simulink model "hdlcoder_ofdm_fft_eml"  (R2026a)
settings: Solver=FixedStepDiscrete  StopTime=5000
PreLoadFcn:
  | wordLength = 12;
  | fracLength = 6;
InitFcn:
  | TotalPoint= 512;
  | TotalStage= 9;
  | FFT_nt=numerictype(1,12, 6);
  | twiddle_Signed = 1;
  | twiddle_WordLength = 12;
  | twiddle_FractionLength = 10;
  | twiddle_nt=numerictype(1,12, 10);
undefined symbols (not defined in the file or in its folder): EbNodB, M, Tsym
libraries: hdlsllib x10, commdigbbndam3 x3, dspxfrm3 x2, commsink2 x2, commchan3 x1, simulink x1, commseqgen3 x1, dspindex x1, commrandsrc3 x1
(part 3 of 3)

== matlab function hdlcoder_ofdm_fft_eml/FFT_512Pt_EML_Serial/Serialized_FFT/FFT_Stages/FFT_Stage9/Control_Logic ==
  settings: fimath=hdlfimath
  data: fft2_x input FFT_nt; fft2_y input FFT_nt; fft2_u output FFT_nt; fft2_v output FFT_nt; twiddle_addr output; enable input boolean; data_in input FFT_nt; index_in input fixdt(0,TotalStage+1,0); data_en output boolean; data_out output FFT_nt; index_out output; mem_rd_dout input FFT_nt; mem_wr_din output FFT_nt; mem_wr_addr output; mem_wr_en output; mem_rd_addr output; TotalStage parameter
function [fft2_u, fft2_v, twiddle_addr, data_en, data_out, index_out, mem_wr_din, mem_wr_addr, mem_wr_en, mem_rd_addr] ...
          = fcn(fft2_x, fft2_y, enable, data_in, index_in, mem_rd_dout, TotalStage)
% FF2 Stages in Serial FFT Model
% Each stage is composed of one FFT2 butterfly computing unit, 
% some memory to cache the streaming data and twiddles, and some control logics.
%
% The incoming streaming data are first stored into cache memory in the data order of last stage,
% and then they are read out in the data order of current stage and send to FFT computing unit.
% The computing unit will produce one result data every clock cycle, and the data_out will streaming
% out the result data in the order of current stage.
% 
% The memory size of each stage is the same as Stage Number, except Stage 1 (the minimum size of
% the memory block is 2). So all the stages share the same code except Stage 1.
% 
% To expand the size of FFT model, user can simply copy and paste new stage blocks and insert them
% before the End_Stage_Reorder block. Only the "Stage" in this code needs to be modified in the new block. 
% And also the size of memory blocks needs to be modified in the new block.
      
Stage = 9;      

N = uint16(2^(Stage-1));
nt = numerictype(data_in);
fm = fimath(data_in);

nt1 = numerictype(0, Stage+1, 0);
nt2 = numerictype(0, Stage-1, 0);
nt3 = numerictype(0, TotalStage-Stage+1, 0);
nt_addr = numerictype(0, TotalStage+1, 0);

% State machine registers
persistent main_state butterfly_state 
nts = numerictype(0, 2, 0);
if isempty(main_state)
    main_state = getfi(0, nts);
end
if isempty(butterfly_state)
    butterfly_state = getfi(0, nts);
end

% Address counters
persistent mem_addr mem_addr1 mem_addr2 
if isempty(mem_addr)
    mem_addr  = getfi(0, nt_addr);
end
if isempty(mem_addr1)
    mem_addr1 = getfi(0, nt_addr);
end
if isempty(mem_addr2)
    mem_addr2 = getfi(0, nt_addr);
end

persistent ctr ctr_lsb1c ctr_lsb2c ctr_msb
if isempty(ctr)
    ctr       = getfi(0, nt1);
end
if isempty(ctr_lsb1c)
    ctr_lsb1c = getfi(0, nt2);
end
if isempty(ctr_lsb2c)
    ctr_lsb2c = getfi(0, nt2);
end
if isempty(ctr_msb)
    ctr_msb   = getfi(0, nt3);
end

% Input/Output
mem_rd_addr  = bitsliceget(mem_addr, Stage, 1);
mem_wr_addr  = bitsliceget(index_in, Stage, 1);
mem_wr_din   = data_in;
index_out    = mem_addr;
twiddle_addr = ctr_lsb1c;

% Delay register inserted before the FFT2 computing unit
persistent reg_u reg_v
if isempty(reg_u)
    reg_u = complex(getfi(0, nt));
end
if isempty(reg_v)
    reg_v = complex(getfi(0, nt));
end
fft2_u = reg_u;
fft2_v = reg_v;

% Main state machine control the memory and data enable signals
switch uint8(main_state)
    case 0 %initial
        mem_wr_en    = false;
        calcu_en     = false;
        data_en      = false;
        ctr_en       = false;
        if enable
            main_state = getfi(1, nts);
        else
            main_state = getfi(0, nts);
        end
        
    case 1 %write data
        mem_wr_en    = true;
        calcu_en     = false;
        data_en      = false;
        ctr_en       = true;
        if ctr == getfi(N-2, nt1)
            main_state = getfi(2, nts);
        else
            main_state = getfi(1, nts);
        end
       
    case 2 %read & calculate data
        mem_wr_en    = true;
        calcu_en     = true;
        data_en      = false;
        ctr_en       = true;
        if ctr == getfi(N+4, nt1)
            main_state = getfi(3, nts);
        else
            main_state = getfi(2, nts);
        end

    case 3 %set output data_en signal, keep calculation
        mem_wr_en    = true;
        calcu_en     = true;
        data_en      = true;
        ctr_en       = false;
        main_state   = getfi(3, nts);
        
    otherwise
        mem_wr_en    = false;
        calcu_en     = false;
        data_en      = false;
        ctr_en       = false;
        main_state   = getfi(0, nts);
end

% Butterfly calculation state machine controls the memory access and data movement
switch uint8(butterfly_state)
    case 0 %initial
        data_out    = fft2_x;
        mem_addr    = mem_addr1;
        ctr_lsb1_en = false;
        ctr_lsb2_en = false;        
        if calcu_en
            butterfly_state = getfi(1, nts);
        else
            butterfly_state = getfi(0, nts);
        end
        
    case 1 %pre-read data
        data_out    = fft2_y;    
        mem_addr    = mem_addr2;
        ctr_lsb1_en = true;
        ctr_lsb2_en = false;
        butterfly_state = getfi(2, nts);

    case 2 %read data -> reg_u
        reg_u       = mem_rd_dout;
        data_out    = fft2_y;
        mem_addr    = mem_addr1;
        ctr_lsb1_en = false;
        ctr_lsb2_en = true;
        butterfly_state = getfi(3, nts);

    case 3 %read data -> reg_v
        reg_v       = mem_rd_dout;       
        data_out    = fft2_x;
        mem_addr    = mem_addr2;
        ctr_lsb1_en = true;
        ctr_lsb2_en = false;
        butterfly_state = getfi(2, nts);   
        
    otherwise
        data_out    = fft2_y;
        mem_addr    = mem_addr1;
        ctr_lsb1_en = false;
        ctr_lsb2_en = false;
        butterfly_state = getfi(0, nts);
end

% Memory address msb counter enable signal
if (ctr_lsb1_en == true) && (ctr_lsb1c == getfi(N-1, nt2))
    ctr_msb_en = true;
else
    ctr_msb_en = false;
end

% Mem_count counter
ctr = update_counter(ctr_en, ctr, nt1);

% Memory address lsb counter 1 
ctr_lsb1c = update_counter(ctr_lsb1_en, ctr_lsb1c, nt2);

% Memory address lsb counter 2
ctr_lsb2c = update_counter(ctr_lsb2_en, ctr_lsb2c, nt2);

% Memory address msb counter
%ctr_msb = update_counter(ctr_msb_en, ctr_msb, nt3);
if ctr_msb_en
    if ctr_msb == getfi(0, nt3)
        ctr_msb = getfi(1, nt3);
    else
        ctr_msb = getfi(0, nt3);
    end    
end

% The output address representation
c0_ufix1 = fi(0, 0, 1, 0, fm);
c1_ufix1 = fi(1, 0, 1, 0, fm);
ctr_lsb1 = bitconcat(c0_ufix1, ctr_lsb1c);
ctr_lsb2 = bitconcat(c1_ufix1, ctr_lsb2c);
mem_addr1 = bitconcat(ctr_msb, ctr_lsb1);
mem_addr2 = bitconcat(ctr_msb, ctr_lsb2);
                  
end

function out = update_counter(enable, in, nt)
if enable
    out = getfi(in + getfi(1, nt), nt);
else
    out = in;
end
end

function f = getfi(u, nt)
f = fi(u, nt, hdlfimath);
end

== matlab function hdlcoder_ofdm_fft_eml/FFT_512Pt_EML_Serial/Serialized_FFT/FFT_Stages/FFT_Stage9/Twiddle_ROM ==
  settings: fimath=hdlfimath
  data: twiddle_addr input; fft2_twiddle output twiddle_nt; TotalPoint parameter; twiddle_Signed parameter; twiddle_WordLength parameter; twiddle_FractionLength parameter
function fft2_twiddle = fcn(twiddle_addr, TotalPoint, twiddle_Signed, twiddle_WordLength, twiddle_FractionLength)
% Twiddle ROM

Stage = 9;

nt = numerictype(twiddle_Signed, twiddle_WordLength, twiddle_FractionLength);
fm = fimath(...
'RoundMode', 'nearest',...
'OverflowMode', 'saturate',...
'ProductMode', 'FullPrecision', 'ProductWordLength', 128,...
'SumMode', 'FullPrecision', 'SumWordLength', 128,...
'CastBeforeSum', true);

% Provide twiddle data for FFT calculation
persistent twiddleValue
if isempty(twiddleValue)
    twiddleValue = fi(exp(-2*pi*1i*(0:(TotalPoint/(2^Stage)):(TotalPoint/2-1))/TotalPoint).', nt, fm);   
end
fft2_twiddle = twiddleValue(int32(twiddle_addr)+1);

== matlab function hdlcoder_ofdm_fft_eml/FFT_512Pt_EML_Serial/Serialized_FFT/Start_Stage_BitReverse/BitReverse_Control_Logics ==
  settings: fimath=hdlfimath
  data: enable input boolean; data_in input FFT_nt; data_en output; data_out output; mem_rd_dout input FFT_nt; mem_wr_din output FFT_nt; mem_wr_addr output; mem_wr_en output; mem_rd_addr output; TotalPoint parameter; TotalStage parameter
function [data_en, data_out, mem_wr_din, mem_wr_addr, mem_wr_en, mem_rd_addr] ...
          = fcn(enable, data_in, mem_rd_dout, TotalPoint, TotalStage)
% Starting Stage -- Bitreverse the order of input serial data
% Memory sized as much as TotalPoint*2 are used to temporary cache the incoming data stream
% The initial delay of this block is fixed as TotalPoint
      
nt = numerictype(data_in);
nt_addr = numerictype(0, TotalStage+1, 0);

% State machines 
persistent main_state
nts = numerictype(0, 2, 0);
if isempty(main_state)
    main_state = getfi(0, nts);
end

% Memory address counters
persistent index_in mem_addr
if isempty(index_in)
    index_in = getfi(0, nt_addr);
end
if isempty(mem_addr)
    mem_addr = getfi(0, nt_addr);
end

% Input/Output
mem_rd_addr = mem_addr;
mem_wr_addr = bitconcat([bitget(index_in, TotalStage+1), bitget(index_in, 1:TotalStage)]);
data_out = mem_rd_dout;

% Delay register for data_in 
persistent reg_data_in
if isempty(reg_data_in)
    reg_data_in = complex(getfi(0, nt));
end

mem_wr_din  = reg_data_in;
reg_data_in = data_in;

switch uint8(main_state)
    case 0 %initial
        mem_wr_en   = false;
        index_in_en = false;
        data_en     = false;
        mem_addr_en = false;        
        if enable
            main_state = getfi(1, nts);
        else
            main_state = getfi(0, nts);
        end
        
    case 1 %write data
        mem_wr_en   = true;
        index_in_en = true;
        data_en     = false;
        mem_addr_en = false;
        if uint16(index_in) == uint16(TotalPoint-47)
            main_state = getfi(2, nts);
        else
            main_state = getfi(1, nts);
        end
       
    case 2 %read data, set data_en for output data
        mem_wr_en   = true;
        index_in_en = true;
        data_en     = true;
        mem_addr_en = true;
        main_state  = getfi(2, nts);
        
    otherwise
        mem_wr_en   = false;
        index_in_en = false;
        data_en     = false;
        mem_addr_en = false;       
        main_state  = getfi(0, nts);
end

% Index_in counter
index_in = update_counter(index_in_en, index_in, nt_addr);

% Memory address counter
mem_addr = update_counter(mem_addr_en, mem_addr, nt_addr);    
end

function out = update_counter(enable, in, nt)
if enable
    out = getfi(in + getfi(1, nt), nt);
else
    out = in;
end
end

function f = getfi(u, nt)
f = fi(u, nt, hdlfimath);
end

== matlab function hdlcoder_ofdm_fft_eml/FFT_512Pt_EML_Serial/Serialized_FFT/FFT_Stages/FFT_Stage2/Butterfly_FFT2_Computing_Unit ==
  settings: fimath=hdlfimath
  data: fft2_u input FFT_nt; fft2_x output FFT_nt; fft2_v input FFT_nt; fft2_twiddle input twiddle_nt; fft2_y output FFT_nt
function [fft2_x, fft2_y] = fcn(fft2_u, fft2_v, fft2_twiddle)
% FFT2 Computing Unit

% Scale down number for this stage. Need to be power of 2.
Scale = 1;

% Call function in hdlcoder_serial_fft_butterfly_scale.m on path 
[x, y] = hdlcoder_serial_fft_butterfly(fft2_u, fft2_v, fft2_twiddle);

% scaling down by 2 for each FFT2 stage.
fft2_x = bitsra(x, log2(Scale));
fft2_y = bitsra(y, log2(Scale));

== matlab function hdlcoder_ofdm_fft_eml/FFT_512Pt_EML_Serial/Serialized_FFT/FFT_Stages/FFT_Stage2/Control_Logic ==
  settings: fimath=hdlfimath
  data: fft2_x input FFT_nt; fft2_y input FFT_nt; fft2_u output FFT_nt; fft2_v output FFT_nt; twiddle_addr output; enable input boolean; data_in input FFT_nt; index_in input fixdt(0,TotalStage+1,0); data_en output boolean; data_out output FFT_nt; index_out output; mem_rd_dout input FFT_nt; mem_wr_din output FFT_nt; mem_wr_addr output; mem_wr_en output; mem_rd_addr output; TotalStage parameter
function [fft2_u, fft2_v, twiddle_addr, data_en, data_out, index_out, mem_wr_din, mem_wr_addr, mem_wr_en, mem_rd_addr] ...
          = fcn(fft2_x, fft2_y, enable, data_in, index_in, mem_rd_dout, TotalStage)
% FF2 Stages in Serial FFT Model
% Each stage is composed of one FFT2 butterfly computing unit, 
% some memory to cache the streaming data and twiddles, and some control logics.
%
% The incoming streaming data are first stored into cache memory in the data order of last stage,
% and then they are read out in the data order of current stage and send to FFT computing unit.
% The computing unit will produce one result data every clock cycle, and the data_out will streaming
% out the result data in the order of current stage.
% 
% The memory size of each stage is the same as Stage Number, except Stage 1 (the minimum size of
% the memory block is 2). So all the stages share the same code except Stage 1.
% 
% To expand the size of FFT model, user can simply copy and paste new stage blocks and insert them
% before the End_Stage_Reorder block. Only the "Stage" in this code needs to be modified in the new block. 
% And also the size of memory blocks needs to be modified in the new block.
      
Stage = 2;      

N = uint16(2^(Stage-1));
nt = numerictype(data_in);
fm = fimath(data_in);

nt1 = numerictype(0, Stage+1, 0);
nt2 = numerictype(0, Stage-1, 0);
nt3 = numerictype(0, TotalStage-Stage+1, 0);
nt_addr = numerictype(0, TotalStage+1, 0);

% State machine registers
persistent main_state butterfly_state 
nts = numerictype(0, 2, 0);
if isempty(main_state)
    main_state = getfi(0, nts);
end
if isempty(butterfly_state)
    butterfly_state = getfi(0, nts);
end

% Address counters
persistent mem_addr mem_addr1 mem_addr2 
if isempty(mem_addr)
    mem_addr  = getfi(0, nt_addr);
end
if isempty(mem_addr1)
    mem_addr1 = getfi(0, nt_addr);
end
if isempty(mem_addr2)
    mem_addr2 = getfi(0, nt_addr);
end

persistent ctr ctr_lsb1c ctr_lsb2c ctr_msb
if isempty(ctr)
    ctr       = getfi(0, nt1);
end
if isempty(ctr_lsb1c)
    ctr_lsb1c = getfi(0, nt2);
end
if isempty(ctr_lsb2c)
    ctr_lsb2c = getfi(0, nt2);
end
if isempty(ctr_msb)
    ctr_msb   = getfi(0, nt3);
end

% Input/Output
mem_rd_addr  = bitsliceget(mem_addr, Stage, 1);
mem_wr_addr  = bitsliceget(index_in, Stage, 1);
mem_wr_din   = data_in;
index_out    = mem_addr;
twiddle_addr = uint8(ctr_lsb1c);

% Delay register inserted before the FFT2 computing unit
persistent reg_u reg_v
if isempty(reg_u)
    reg_u = complex(getfi(0, nt));
end
if isempty(reg_v)
    reg_v = complex(getfi(0, nt));
end
fft2_u = reg_u;
fft2_v = reg_v;

% Main state machine control the memory and data enable signals
switch uint8(main_state)
    case 0 %initial
        mem_wr_en    = false;
        calcu_en     = false;
        data_en      = false;
        ctr_en       = false;
        if enable
            main_state = getfi(1, nts);
        else
            main_state = getfi(0, nts);
        end
        
    case 1 %write data
        mem_wr_en    = true;
        calcu_en     = false;
        data_en      = false;
        ctr_en       = true;
        if ctr == getfi(N-2, nt1)
            main_state = getfi(2, nts);
        else
            main_state = getfi(1, nts);
        end
       
    case 2 %read & calculate data
        mem_wr_en    = true;
        calcu_en     = true;
        data_en      = false;
        ctr_en       = true;
        if ctr == getfi(N+4, nt1)
            main_state = getfi(3, nts);
        else
            main_state = getfi(2, nts);
        end

    case 3 %set output data_en signal, keep calculation
        mem_wr_en    = true;
        calcu_en     = true;
        data_en      = true;
        ctr_en       = false;
        main_state   = getfi(3, nts);
        
    otherwise
        mem_wr_en    = false;
        calcu_en     = false;
        data_en      = false;
        ctr_en       = false;
        main_state   = getfi(0, nts);
end

% Butterfly calculation state machine controls the memory access and data movement
switch uint8(butterfly_state)
    case 0 %initial
        data_out    = fft2_x;
        mem_addr    = mem_addr1;
        ctr_lsb1_en = false;
        ctr_lsb2_en = false;        
        if calcu_en
            butterfly_state = getfi(1, nts);
        else
            butterfly_state = getfi(0, nts);
        end
        
    case 1 %pre-read data
        data_out    = fft2_y;    
        mem_addr    = mem_addr2;
        ctr_lsb1_en = true;
        ctr_lsb2_en = false;
        butterfly_state = getfi(2, nts);

    case 2 %read data -> reg_u
        reg_u       = mem_rd_dout;
        data_out    = fft2_y;
        mem_addr    = mem_addr1;
        ctr_lsb1_en = false;
        ctr_lsb2_en = true;
        butterfly_state = getfi(3, nts);

    case 3 %read data -> reg_v
        reg_v       = mem_rd_dout;       
        data_out    = fft2_x;
        mem_addr    = mem_addr2;
        ctr_lsb1_en = true;
        ctr_lsb2_en = false;
        butterfly_state = getfi(2, nts);   
        
    otherwise
        data_out    = fft2_y;
        mem_addr    = mem_addr1;
        ctr_lsb1_en = false;
        ctr_lsb2_en = false;
        butterfly_state = getfi(0, nts);
end

% Memory address msb counter enable signal
if (ctr_lsb1_en == true) && (ctr_lsb1c == getfi(N-1, nt2))
    ctr_msb_en = true;
else
    ctr_msb_en = false;
end

% Mem_count counter
ctr = update_counter(ctr_en, ctr, nt1);

% Memory address lsb counter 1 
%ctr_lsb1c = update_counter(ctr_lsb1_en, ctr_lsb1c, nt2);
if ctr_lsb1_en == true
    if ctr_lsb1c == getfi(0, nt2)
        ctr_lsb1c = getfi(1, nt2);
    else
        ctr_lsb1c = getfi(0, nt2);
    end
end

% Memory address lsb counter 2
%ctr_lsb2c = update_counter(ctr_lsb2_en, ctr_lsb2c, nt2);
if ctr_lsb2_en
    if ctr_lsb2c == getfi(0, nt2)
        ctr_lsb2c = getfi(1, nt2);
    else
        ctr_lsb2c = getfi(0, nt2);
    end
end

% Memory address msb counter
ctr_msb = update_counter(ctr_msb_en, ctr_msb, nt3);

% The output address representation
c0_ufix1 = fi(0, 0, 1, 0, fm);
c1_ufix1 = fi(1, 0, 1, 0, fm);
ctr_lsb1 = bitconcat(c0_ufix1, ctr_lsb1c);
ctr_lsb2 = bitconcat(c1_ufix1, ctr_lsb2c);
mem_addr1 = bitconcat(ctr_msb, ctr_lsb1);
mem_addr2 = bitconcat(ctr_msb, ctr_lsb2);
                  
end

function out = update_counter(enable, in, nt)
if enable
    out = getfi(in + getfi(1, nt), nt);
else
    out = in;
end
end

function f = getfi(u, nt)
f = fi(u, nt, hdlfimath);
end

== matlab function hdlcoder_ofdm_fft_eml/FFT_512Pt_EML_Serial/Serialized_FFT/FFT_Stages/FFT_Stage2/Twiddle_ROM ==
  settings: fimath=hdlfimath
  data: twiddle_addr input; fft2_twiddle output twiddle_nt; TotalPoint parameter; twiddle_Signed parameter; twiddle_WordLength parameter; twiddle_FractionLength parameter
function fft2_twiddle = fcn(twiddle_addr, TotalPoint, twiddle_Signed, twiddle_WordLength, twiddle_FractionLength)
% Twiddle ROM

Stage = 2;

nt = numerictype(twiddle_Signed, twiddle_WordLength, twiddle_FractionLength);
fm = fimath(...
'RoundMode', 'nearest',...
'OverflowMode', 'saturate',...
'ProductMode', 'FullPrecision', 'ProductWordLength', 128,...
'SumMode', 'FullPrecision', 'SumWordLength', 128,...
'CastBeforeSum', true);

% Provide twiddle data for FFT calculation
persistent twiddleValue
if isempty(twiddleValue)
    twiddleValue = fi(exp(-2*pi*1i*(0:(TotalPoint/(2^Stage)):(TotalPoint/2-1))/TotalPoint).', nt, fm);   
end
fft2_twiddle = twiddleValue(int32(twiddle_addr)+1);
